simulink model "QD2_MissionCtrl_NoJoystick_2021a"  (R2022a)
settings: Solver=ode2  StartTime=0.0  StopTime=inf  FixedStep=0.001  RelTol=1e-3  EnableMultiTasking=on
undefined symbols (not defined in the file or in its folder): _MissionCtrl, datetime, Host, localhost, log_, m, qc_get_step_size, saved_data
libraries: quarc_library x30, simulink x7
(part 2 of 2)

== system QD2_MissionCtrl_NoJoystick_2021a/MISSION CONTROL QDRONE POSITION CONTROL/Localization - Vicon/For Each Subsystem (Convention Correction: Vicon Frame to Research Studio Frame)/Prevent Gimbal Lock ==
  Attitude in MF (rad) [3] : Inport
  Demux : Demux  Outputs=3
  Euler Angles from Rotation Matrix (Relative ZYX) : quarc_library/Math Operations/Matrices/Euler Angles from Rotation Matrix  menu_order=Relative Z-Y-X
      settings: SourceProductName=QUARC Targets
  Euler Angles to Rotation Matrix (Relative XYZ) : quarc_library/Math Operations/Matrices/Euler Angles to Rotation Matrix  menu_order=Relative X-Y-Z
      settings: SourceProductName=QUARC Targets
  Mux : Mux  Inputs=3
  Quaternion from Rotation Matrix : quarc_library/Math Operations/Quaternions/Quaternion from Rotation Matrix
      settings: SourceProductName=QUARC Targets
  Attitude in RSF (rad) [3] : Outport
  q [4] : Outport  Port=2
  wires:
  Euler Angles to Rotation Matrix (Relative XYZ)/1 -> Quaternion from Rotation Matrix/1, Euler Angles from Rotation Matrix (Relative ZYX)/1
  Euler Angles from Rotation Matrix (Relative ZYX)/3 -> Mux/1
  Euler Angles from Rotation Matrix (Relative ZYX)/2 -> Mux/2
  Euler Angles from Rotation Matrix (Relative ZYX)/1 -> Mux/3
  Mux/1 -> Attitude in RSF (rad) [3]/1
  Demux/1 -> Euler Angles to Rotation Matrix (Relative XYZ)/3
  Demux/3 -> Euler Angles to Rotation Matrix (Relative XYZ)/2
  Demux/2 -> Euler Angles to Rotation Matrix (Relative XYZ)/1
  Attitude in MF (rad) [3]/1 -> Demux/1
  Quaternion from Rotation Matrix/1 -> q [4]/1

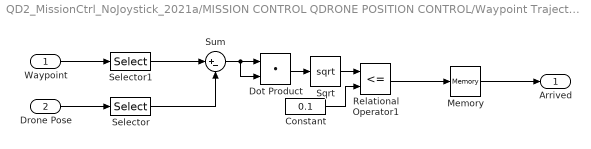
== system QD2_MissionCtrl_NoJoystick_2021a/MISSION CONTROL QDRONE POSITION CONTROL/Waypoint Trajectories/Waypoint_Generator/Arrived ==
  Waypoint : Inport
  Drone Pose : Inport  Port=2
  Constant : Constant  Value=0.1
  Dot Product : DotProduct  OutDataTypeStr=Inherit: Inherit via internal rule
  Memory : Memory
  Relational Operator1 : RelationalOperator  Operator=<=  OutDataTypeStr=boolean  InputSameDT=off
  Selector : Selector  InputPortWidth=4  IndexOptions=Index vector (dialog)  Indices=[1 2]  OutputSizes=1
  Selector1 : Selector  InputPortWidth=4  IndexOptions=Index vector (dialog)  Indices=[1 2]  OutputSizes=1
  Sqrt : Sqrt
  Sum : Sum  Inputs=|+-
  Arrived : Outport
  wires:
  Sum/1 -> Dot Product/2, Dot Product/1
  Selector1/1 -> Sum/1
  Selector/1 -> Sum/2
  Constant/1 -> Relational Operator1/2
  Relational Operator1/1 -> Memory/1
  Dot Product/1 -> Sqrt/1
  Memory/1 -> Arrived/1
  Sqrt/1 -> Relational Operator1/1
  Drone Pose/1 -> Selector/1
  Waypoint/1 -> Selector1/1

== system QD2_MissionCtrl_NoJoystick_2021a/MISSION CONTROL QDRONE POSITION CONTROL/Waypoint Trajectories/Waypoint_Generator/Timer ==
  Wait time : Inport
  arrived : Inport  Port=2
  Cast To Double : DataTypeConversion  OutDataTypeStr=double  SaturateOnIntegerOverflow=off  RndMeth=Floor
  "Detect Rise Positive " : simulink/Logic and Bit Operations/Detect Rise Positive  vinit=0  OutDataTypeStr=boolean
  GreaterThan : RelationalOperator  Operator=<  OutDataTypeStr=boolean  RndMeth=Simplest  InputSameDT=off
  Integrator : Integrator  ExternalReset=falling
  Mux : Mux  Inputs=2
  Scope : Scope
  trigger : Outport
  wires:
  Integrator/1 -> GreaterThan/2
  Wait time/1 -> GreaterThan/1
  arrived/1 -> Cast To Double/1, Mux/2, Integrator/2
  GreaterThan/1 -> "Detect Rise Positive "/1
  Cast To Double/1 -> Integrator/1
  Mux/1 -> Scope/1
  "Detect Rise Positive "/1 -> trigger/1, Mux/1

== matlab function QD2_MissionCtrl_NoJoystick_2021a/MISSION CONTROL QDRONE POSITION CONTROL/Subsystem/MATLAB Function ==
  data: Arm input; Flight_State output; Takeoff_Land_Flag input; Emergency_Stop input; Joystick_Issue input; Stop_MS output; Communication_Issue input
function [Flight_State, Stop_MS]= Flight_Plan(Arm, ...
                            Takeoff_Land_Flag, ...
                            Emergency_Stop, ...
                            Joystick_Issue, ...
                            Communication_Issue)

persistent State

if isempty(State);
    State = 0;

end 
Stop_MS = 0;


switch State 

    case 0 % ============== QDrone Idle Sate ============== 
            
        if  Arm == 1 & Emergency_Stop == 0 && Joystick_Issue == 0
            State = 1;
        elseif Joystick_Issue == 1 || Emergency_Stop == 1 || Takeoff_Land_Flag == 1 || Communication_Issue == 1
            State = 9 ;
        end 

    case 1 % ============== QDrone Armed Sate ============== 
          if Emergency_Stop == 0 && Joystick_Issue == 0 
               if Arm == 0 
                     State = 0 ;
               elseif Arm == 1 && Takeoff_Land_Flag == 1 
                     State = 2 ;
                 end
              elseif Joystick_Issue == 1 || Communication_Issue == 1 || Emergency_Stop == 1
                State = 9 ;
        end 
          
    case 2 % ============== QDrone Takeoff Sate ============== 
          if Emergency_Stop == 0 && Joystick_Issue == 0 
               if Takeoff_Land_Flag == 0 
                State = 3 ;
              elseif Joystick_Issue == 1 || Arm == 0 || Communication_Issue == 1|| Emergency_Stop == 1
                State = 9 ;
               end 
          end 

    case 3 % ============== QDrone Land Sate ============== 
           if Joystick_Issue == 1 || Arm == 0 || Communication_Issue == 1
               State = 9 ;
           end

    case 9 % ============== MS Stop Sate ============== 
            Stop_MS = 1;
    
end 

Flight_State = State ;

== matlab function QD2_MissionCtrl_NoJoystick_2021a/Communication/Detect Communication loss/MATLAB Function ==
  data: time input; stream_connection_loss output; state input; error input
function stream_connection_loss  = fcn(time, state, error)

stream_connection_loss = 0;
if time > 1
    if ~((state == 2)&&(error >= 0))
        % stream connection is not established correctly
        stream_connection_loss = 1;
    end
end

== matlab function QD2_MissionCtrl_NoJoystick_2021a/MISSION CONTROL QDRONE POSITION CONTROL/Waypoint Trajectories/Waypoint_Generator/MATLAB Function ==
  data: waypoints_0 input; waypoint output; trigger input; finished output
function [waypoint, finished]  = fcn(waypoints_0, trigger)
persistent idx status;
[m, ~] = size(waypoints_0);
finished = 0;
if isempty(idx)
    idx = 1;
    status = 0;
    
end

if trigger && idx < m && status == 0 
    idx = idx + 1;
end     
if  trigger && idx == m
    
    status = 1; 
    finished =1;
end 

waypoint = waypoints_0(idx, :);
